simulink model "mobile_manipulator_variant"  (R2025b)
settings: Solver=ode15s  StartTime=0.0  StopTime=10  RelTol=1e-3
libraries: sm_lib x7, nesl_utility x5
settings Model: Creator=SIDHANT  LastModifiedBy=SIDHANT

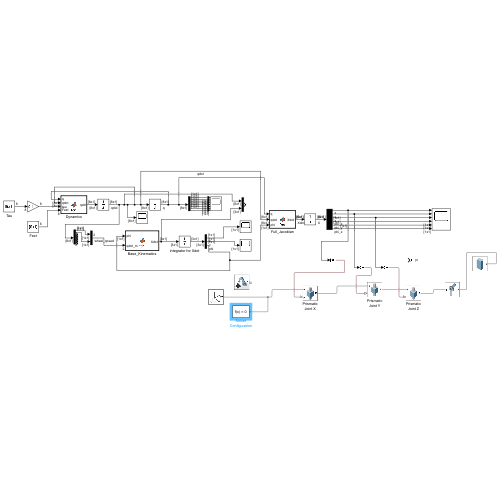
[thumbnail: Simulink's stored preview of the top-level diagram]
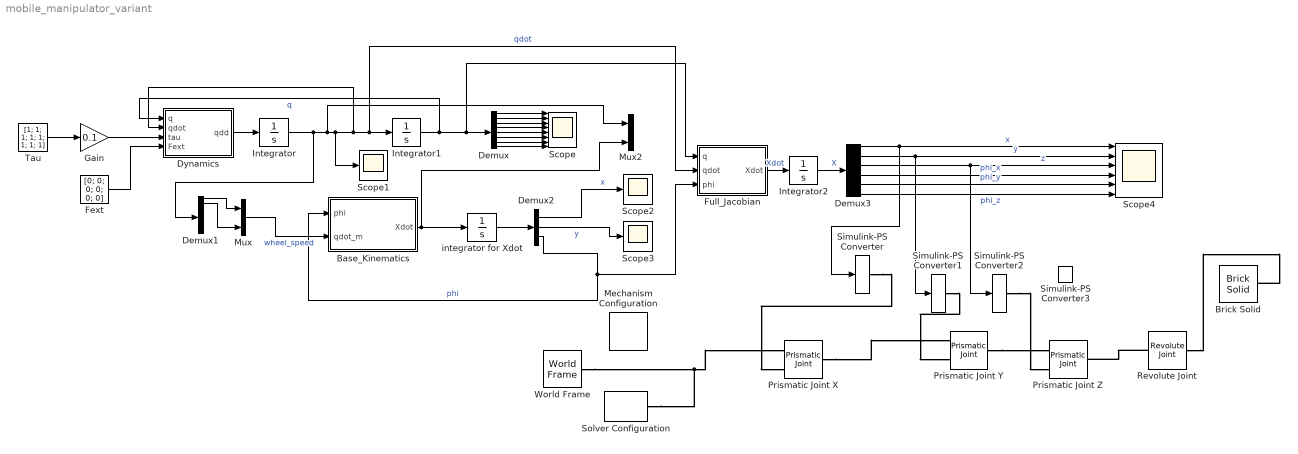
== system mobile_manipulator_variant ==
  Base_Kinematics : MATLAB Function  TreatAsAtomicUnit=on
  Brick Solid : sm_lib/Body Elements/Brick Solid  BrickDimensions=[0.3 0.2 0.1]  BrickDimensionsUnits=m  ExportEntireGeometry=off  InertiaType=CalculateFromGeometry  BasedOnType=Density  Density=1000  DensityUnits=kg/m^3  Mass=1  MassUnits=kg  CenterOfMass=[0 0 0]  CenterOfMassUnits=m  MomentsOfInertia=[1 1 1]  MomentsOfInertiaUnits=kg*m^2  ProductsOfInertia=[0 0 0]  ProductsOfInertiaUnits=kg*m^2  GraphicType=FromGeometry  MarkerShape=Sphere  MarkerSize=10  GraphicVisPropType=SimpleVisualProperties  GraphicDiffuseColor=[0.5 0.5 0.5]  GraphicOpacity=1  GraphicSpecularColor=[0.5 0.5 0.5 1.0]  GraphicAmbientColor=[0.15 0.15 0.15 1.0]  GraphicEmissiveColor=[0.0 0.0 0.0 1.0]  GraphicShininess=75  DoExposeReferenceFrame=on  SerializedFrames=<Frames/>
  Demux : Demux  Outputs=8
  Demux1 : Demux  Outputs=8
  Demux2 : Demux  Outputs=3
  Demux3 : Demux  Outputs=6
  Dynamics : MATLAB Function  TreatAsAtomicUnit=on
  Fext : Constant  Value=[0; 0; 0; 0; 0; 0]
  Full_Jacobian : MATLAB Function  TreatAsAtomicUnit=on
  Gain : Gain  Gain=0.1
  Integrator : Integrator  InitialCondition=zeros(8,1)
  Integrator1 : Integrator  InitialCondition=zeros(8,1)
  Integrator2 : Integrator  InitialCondition=zeros(6,1)
  Mechanism Configuration : sm_lib/Utilities/Mechanism Configuration  UniformGravity=Constant  GravityVector=[0 0 -9.80665]  GravityVectorUnits=m/s^2  LinearizationDelta=0.001  JointModeTransitionNonlinearIterations=2
  Mux : Mux  Inputs=2
  Mux2 : Mux  Inputs=2
  Prismatic Joint X : sm_lib/Joints/Prismatic Joint  JointMode=Normal  CompositeWrenchDir=FollowerOnBase  CompositeWrenchFrame=BaseFrame  SenseConstraintForce=off  SenseConstraintTorque=off  SenseTotalForce=off  SenseTotalTorque=off  PositionTargetSpecify=off  PositionTargetPriority=High  PositionTargetValue=0  PositionTargetValueUnits=m  VelocityTargetSpecify=off  VelocityTargetPriority=High  VelocityTargetValue=0  VelocityTargetValueUnits=m/s  EquilibriumPosition=0  EquilibriumPositionUnits=m  SpringStiffness=0  SpringStiffnessUnits=N/m  DampingCoefficient=0  DampingCoefficientUnits=N/(m/s)  LowerLimitSpecify=off  LowerLimitBound=-1  LowerLimitBoundUnits=m  LowerLimitStiffness=1e6  LowerLimitStiffnessUnits=N/m  LowerLimitDamping=1e3  LowerLimitDampingUnits=N/(m/s)  LowerLimitTransitionRegionWidth=1e-4  LowerLimitTransitionRegionWidthUnits=m  UpperLimitSpecify=off  UpperLimitBound=1  UpperLimitBoundUnits=m  UpperLimitStiffness=1e6  UpperLimitStiffnessUnits=N/m  UpperLimitDamping=1e3  UpperLimitDampingUnits=N/(m/s)  UpperLimitTransitionRegionWidth=1e-4  UpperLimitTransitionRegionWidthUnits=m  TorqueActuationMode=ComputedTorque  MotionActuationMode=InputMotion  SensePosition=off  SenseVelocity=off  SenseAcceleration=off  SenseTorqueForce=off  SenseLowerLimitTorqueForce=off  SenseUpperLimitTorqueForce=off
  Prismatic Joint Y : sm_lib/Joints/Prismatic Joint  JointMode=Normal  CompositeWrenchDir=FollowerOnBase  CompositeWrenchFrame=BaseFrame  SenseConstraintForce=off  SenseConstraintTorque=off  SenseTotalForce=off  SenseTotalTorque=off  PositionTargetSpecify=off  PositionTargetPriority=High  PositionTargetValue=0  PositionTargetValueUnits=m  VelocityTargetSpecify=off  VelocityTargetPriority=High  VelocityTargetValue=0  VelocityTargetValueUnits=m/s  EquilibriumPosition=0  EquilibriumPositionUnits=m  SpringStiffness=0  SpringStiffnessUnits=N/m  DampingCoefficient=0  DampingCoefficientUnits=N/(m/s)  LowerLimitSpecify=off  LowerLimitBound=-1  LowerLimitBoundUnits=m  LowerLimitStiffness=1e6  LowerLimitStiffnessUnits=N/m  LowerLimitDamping=1e3  LowerLimitDampingUnits=N/(m/s)  LowerLimitTransitionRegionWidth=1e-4  LowerLimitTransitionRegionWidthUnits=m  UpperLimitSpecify=off  UpperLimitBound=1  UpperLimitBoundUnits=m  UpperLimitStiffness=1e6  UpperLimitStiffnessUnits=N/m  UpperLimitDamping=1e3  UpperLimitDampingUnits=N/(m/s)  UpperLimitTransitionRegionWidth=1e-4  UpperLimitTransitionRegionWidthUnits=m  TorqueActuationMode=ComputedTorque  MotionActuationMode=InputMotion  SensePosition=off  SenseVelocity=off  SenseAcceleration=off  SenseTorqueForce=off  SenseLowerLimitTorqueForce=off  SenseUpperLimitTorqueForce=off
  Prismatic Joint Z : sm_lib/Joints/Prismatic Joint  JointMode=Normal  CompositeWrenchDir=FollowerOnBase  CompositeWrenchFrame=BaseFrame  SenseConstraintForce=off  SenseConstraintTorque=off  SenseTotalForce=off  SenseTotalTorque=off  PositionTargetSpecify=off  PositionTargetPriority=High  PositionTargetValue=0  PositionTargetValueUnits=m  VelocityTargetSpecify=off  VelocityTargetPriority=High  VelocityTargetValue=0  VelocityTargetValueUnits=m/s  EquilibriumPosition=0  EquilibriumPositionUnits=m  SpringStiffness=0  SpringStiffnessUnits=N/m  DampingCoefficient=0  DampingCoefficientUnits=N/(m/s)  LowerLimitSpecify=off  LowerLimitBound=-1  LowerLimitBoundUnits=m  LowerLimitStiffness=1e6  LowerLimitStiffnessUnits=N/m  LowerLimitDamping=1e3  LowerLimitDampingUnits=N/(m/s)  LowerLimitTransitionRegionWidth=1e-4  LowerLimitTransitionRegionWidthUnits=m  UpperLimitSpecify=off  UpperLimitBound=1  UpperLimitBoundUnits=m  UpperLimitStiffness=1e6  UpperLimitStiffnessUnits=N/m  UpperLimitDamping=1e3  UpperLimitDampingUnits=N/(m/s)  UpperLimitTransitionRegionWidth=1e-4  UpperLimitTransitionRegionWidthUnits=m  TorqueActuationMode=ComputedTorque  MotionActuationMode=InputMotion  SensePosition=off  SenseVelocity=off  SenseAcceleration=off  SenseTorqueForce=off  SenseLowerLimitTorqueForce=off  SenseUpperLimitTorqueForce=off
  Revolute Joint : sm_lib/Joints/Revolute Joint  JointMode=Normal  CompositeWrenchDir=FollowerOnBase  CompositeWrenchFrame=BaseFrame  SenseConstraintForce=off  SenseConstraintTorque=off  SenseTotalForce=off  SenseTotalTorque=off  PositionTargetSpecify=off  PositionTargetPriority=High  PositionTargetValue=0  PositionTargetValueUnits=deg  VelocityTargetSpecify=off  VelocityTargetPriority=High  VelocityTargetValue=0  VelocityTargetValueUnits=deg/s  EquilibriumPosition=0  EquilibriumPositionUnits=deg  SpringStiffness=0  SpringStiffnessUnits=N*m/deg  DampingCoefficient=0  DampingCoefficientUnits=N*m/(deg/s)  LowerLimitSpecify=off  LowerLimitBound=-90  LowerLimitBoundUnits=deg  LowerLimitStiffness=1e4  LowerLimitStiffnessUnits=N*m/deg  LowerLimitDamping=10  LowerLimitDampingUnits=N*m/(deg/s)  LowerLimitTransitionRegionWidth=0.1  LowerLimitTransitionRegionWidthUnits=deg  UpperLimitSpecify=off  UpperLimitBound=90  UpperLimitBoundUnits=deg  UpperLimitStiffness=1e4  UpperLimitStiffnessUnits=N*m/deg  UpperLimitDamping=10  UpperLimitDampingUnits=N*m/(deg/s)  UpperLimitTransitionRegionWidth=0.1  UpperLimitTransitionRegionWidthUnits=deg  TorqueActuationMode=NoTorque  MotionActuationMode=ComputedMotion  SensePosition=off  SenseVelocity=off  SenseAcceleration=off  SenseTorqueForce=off  SenseLowerLimitTorqueForce=off  SenseUpperLimitTorqueForce=off
  Scope : Scope  NumInputPorts=8
      settings: ActiveDisplayYMinimum=-2.0517386444935086  ActiveDisplayYMaximum=27.497370231287729
  Scope1 : Scope
      settings: ActiveDisplayYMinimum=-1  ActiveDisplayYMaximum=1
  Scope2 : Scope
      settings: DataLoggingVariableName=ScopeData2
  Scope3 : Scope
      settings: DataLoggingVariableName=ScopeData3
  Scope4 : Scope  NumInputPorts=6
      settings: ActiveDisplayYMinimum=-0.6937817624720295  ActiveDisplayYMaximum=0.80747157145308834  DataLoggingVariableName=ScopeData4
  Simulink-PS Converter : nesl_utility/Simulink-PS Converter  PhysicalDomain=network_engine_domain  SubClassName=ps_input  LeftPortType=input  RightPortType=output  PseudoPeriodic=off  Frequencies=[]  NoiseDistribution=none  NoiseParameters=[]  Unit=m  AffineConversion=off  FilteringAndDerivatives=filter  SimscapeFilterOrder=1  InputFilterTimeConstant=0.001  UdotUserProvided=2
  Simulink-PS Converter1 : nesl_utility/Simulink-PS Converter  PhysicalDomain=network_engine_domain  SubClassName=ps_input  LeftPortType=input  RightPortType=output  PseudoPeriodic=off  Frequencies=[]  NoiseDistribution=none  NoiseParameters=[]  Unit=m  AffineConversion=off  FilteringAndDerivatives=filter  SimscapeFilterOrder=1  InputFilterTimeConstant=0.001  UdotUserProvided=2
  Simulink-PS Converter2 : nesl_utility/Simulink-PS Converter  PhysicalDomain=network_engine_domain  SubClassName=ps_input  LeftPortType=input  RightPortType=output  PseudoPeriodic=off  Frequencies=[]  NoiseDistribution=none  NoiseParameters=[]  Unit=m  AffineConversion=off  FilteringAndDerivatives=filter  SimscapeFilterOrder=1  InputFilterTimeConstant=0.001  UdotUserProvided=2
  Simulink-PS Converter3 : nesl_utility/Simulink-PS Converter  PhysicalDomain=network_engine_domain  SubClassName=ps_input  LeftPortType=input  RightPortType=output  PseudoPeriodic=off  Frequencies=[]  NoiseDistribution=none  NoiseParameters=[]  Unit=rad  AffineConversion=off  FilteringAndDerivatives=provide  SimscapeFilterOrder=1  InputFilterTimeConstant=0.001  UdotUserProvided=0
  Solver Configuration : nesl_utility/Solver Configuration  PhysicalDomain=network_engine_domain  SubClassName=solver  LeftPortType=input  RightPortType=generic  Tones=[]  Harmonics=[]  SimulateNoise=off  Profile=off  UseLocalSampling=off  EnableSwitchedLinearOptims=on  FrequencyDomain=off  UseCCode=off  RelTol=0.001  AbsTol=0.001  MinStep=1e-09  ToWorkspace=off  RevertToSquareIcSolve=off  NumHomotopyIterations=100  PhasorMode=off  PhasorModeNumHarmonics=1  ConsistencySolver=NEWTON_XTOL_AFTER_FTOL  IndexReductionMethod=DerivativeReplacement  DoDC=off  ResidualTolerance=1e-09  ConsistencyTolSource=GLOBAL  ConsistencyAbsTol=0.001  ConsistencyRelTol=0.001  ConsistencyTolFactor=0.001  UseLocalSolver=off  LocalSolverChoice=NE_BACKWARD_EULER_ADVANCER  ResolveIndetEquations=on  FunctionEvalNumThread=1  LocalSolverSampleTime=0.001  DoFixedCost=off  MaxNonlinIter=3  MaxModeIter=2  ComputeImpulses=off  ImpulseIterations=2  LinearAlgebra=auto  LinearAlgebraNumThread=0  EquationFormulation=NE_TIME_EF  DelaysMemoryBudget=1024  AutomaticFiltering=on  FilteringTimeConstant=0.001  PartitionStorageMethod=AS_NEEDED  PartitionMemoryBudget=1024  PartitionMethod=ROBUST  MultibodyUseLocalSolver=off  MultibodyLocalSolverChoice=ODE1  MultibodyLocalSolverSampleTime=0.001
  Tau : Constant  Value=[1; 1; 1; 1; 1; 1; 1; 1]
  World Frame : sm_lib/Frames and Transforms/World Frame
  integrator for Xdot : Integrator  InitialCondition=[0;0;0]
  wires:
  Dynamics/1(qdd) -> Integrator/1
  Integrator1/1 -> Full_Jacobian/1(q), Demux/1, Dynamics/1(q)  "q"
  Fext/1 -> Dynamics/4(Fext)
  Demux/5 -> Scope/5
  Demux/6 -> Scope/6
  Demux/8 -> Scope/8
  Demux/7 -> Scope/7
  Demux/4 -> Scope/4
  Demux/3 -> Scope/3
  Demux/2 -> Scope/2
  Demux/1 -> Scope/1
  Integrator/1 -> Demux1/1, Mux2/1, Full_Jacobian/2(qdot), Integrator1/1, Dynamics/2(qdot), Scope1/1  "qdot"
  Demux1/1 -> Mux/1
  Demux1/2 -> Mux/2
  Base_Kinematics/1(Xdot) -> integrator for Xdot/1, Mux2/2
  Mux/1 -> Base_Kinematics/2(qdot_m)  "wheel_speed"
  integrator for Xdot/1 -> Demux2/1
  Demux2/3 -> Base_Kinematics/1(phi), Full_Jacobian/3(phi)  "phi"
  Demux2/1 -> Scope2/1  "x"
  Demux2/2 -> Scope3/1  "y"
  Full_Jacobian/1(Xdot) -> Integrator2/1  "Xdot"
  Integrator2/1 -> Demux3/1  "X"
  Demux3/1 -> Simulink-PS Converter/1, Scope4/1  "x"
  Demux3/2 -> Scope4/2, Simulink-PS Converter1/1  "y"
  Demux3/3 -> Simulink-PS Converter2/1, Scope4/3  "z"
  Demux3/4 -> Scope4/4  "phi_x"
  Demux3/5 -> Scope4/5  "phi_y"
  Demux3/6 -> Scope4/6  "phi_z"
  Tau/1 -> Gain/1
  Gain/1 -> Dynamics/3(tau)
  connections:
  Prismatic Joint Y/RConn1 -- Prismatic Joint Z/LConn1
  Revolute Joint/LConn1 -- Prismatic Joint Z/RConn1
  Revolute Joint/RConn1 -- Brick Solid/RConn1
  Simulink-PS Converter1/RConn1 -- Prismatic Joint Y/LConn2
  Simulink-PS Converter2/RConn1 -- Prismatic Joint Z/LConn2
  Simulink-PS Converter/RConn1 -- Prismatic Joint X/LConn2
  Prismatic Joint X/RConn1 -- Prismatic Joint Y/LConn1
  World Frame/RConn1 -- Solver Configuration/RConn1 -- Prismatic Joint X/LConn1

== matlab function mobile_manipulator_variant/Base_Kinematics ==
  data: phi input; Xdot output; qdot_m input
function Xdot = fcn(phi, qdot_m)

r = 0.1;
L = 0.5;

thetaR = qdot_m(1);
thetaL = qdot_m(2);

% Jacobian
J = [ (r/2)*cos(phi),  (r/2)*cos(phi);
      (r/2)*sin(phi),  (r/2)*sin(phi);
      (r/(2*L)),       -(r/(2*L)) ];

% Joint velocity vector
qdot_vec = [thetaR; thetaL];

% Final equation
Xdot = J * qdot_vec;

end

== matlab function mobile_manipulator_variant/Dynamics ==
  data: q input; qdd output; qdot input; tau input; Fext input
function qdd = fcn(q, qdot, tau, Fext)

n = 8;   % 2 wheels + 6 joints

% ===== TEMP (we replace later with your real equations) =====
M = eye(n);
C = zeros(n);
G = zeros(n,1);

% Full Jacobian (6x8)
J = zeros(6,8);   % from your PDF

% External force mapping
tau_ext = J' * Fext;

% Dynamics
qdd = M \ (tau - tau_ext - C*qdot - G);

end

== matlab function mobile_manipulator_variant/Full_Jacobian ==
  data: q input; Xdot output; qdot input; phi input
function Xdot = fcn(q, qdot, phi)

r = 0.1;
L = 0.5;

%% BASE PART
thetaR_dot = qdot(1);
thetaL_dot = qdot(2);

Jm = (r/2)*[
    cos(phi) cos(phi);
    sin(phi) sin(phi);
    0 0;
    0 0;
    0 0;
    1/L -1/L
];

Xdot_base = Jm * [thetaR_dot; thetaL_dot];

%% ARM PART
qdot_a = qdot(3:8);
theta = q(3:8);

t1 = theta(1);
t2 = theta(2);
t3 = theta(3);
t4 = theta(4);
t5 = theta(5);
t6 = theta(6);

l1 = 0.5;
l2 = 0.4;
l3 = 0.3;

Jv = [
    -l2*sin(t1+t2) - l3*sin(t1+t2+t3),   -l2*sin(t1+t2) - l3*sin(t1+t2+t3),   -l3*sin(t1+t2+t3),   0 0 0;
     l2*cos(t1+t2) + l3*cos(t1+t2+t3),    l2*cos(t1+t2) + l3*cos(t1+t2+t3),    l3*cos(t1+t2+t3),   0 0 0;
     l1,                                   l1,                                   l1,                0 0 0
];

Jw = [
    0 0 0 1 0 0;
    0 0 0 0 1 0;
    1 1 1 0 0 1
];

Ja = [Jv;
      Jw];

Xdot_arm = Ja * qdot_a;

%% TOTAL
J = [Jm, Ja];   % 6x8

Xdot = J * qdot;

end
